simulink model "turbo_controller"  (R2025a)
settings: Solver=FixedStepAuto  StartTime=0.0  StopTime=inf  FixedStep=0.001  RelTol=1e-3
PostLoadFcn:
  | % 自动定位同目录CubeMX文件；不需要外部初始化脚本。
  | codertarget.data.setParameterValue('turbo_controller','STM32CubeMX.ProjectFile',fullfile(fileparts(get_param('turbo_controller','FileName')),'turbo_f407.ioc'));
InitFcn:
  | % 中文说明：按原控制器字段与类型创建三组接口总线；控制参数已内嵌。
  | tc_names=["EValve_Cycle" "EValve_Open" "Eblast_Cycle" "Eblast_Open" "Motor_Cycle" "Motor_Open" "EValve_Enable" "Eblast_Enable" "Motor_Enable" "SWO_Firework" "SWO_BleedAir" "EngineState" "Flag_ECUReset_Clear" "Flag_ECUReset_Save" "Flag_Reset_Enable" "Accelerator" "Nc_dem" "Nc"]; tc_types=["uint16" "uint16" "uint16" "uint16" "uint16" "uint16" "uint8" "uint8" "uint8" "uint8" "uint8" "uint8" "uint8" "uint8" "uint8" "single" "single" "single"];
  | for tc_k=1:numel(tc_names)
  |  tc_e(tc_k)=Simulink.BusElement; tc_e(tc_k).Name=char(tc_names(tc_k)); tc_e(tc_k).DataType=char(tc_types(tc_k));
  | end
  | EngineControl_Out=Simulink.Bus; EngineControl_Out.DataScope='Exported'; EngineControl_Out.Elements=tc_e;
  | clear tc_e tc_names tc_types tc_k
  | tc_names=["savedata1" "savedata2" "savedata3" "savedata4" "savedata5" "savedata6" "savedata7" "savedata8" "savedata9" "savedata10" "savedata11" "savedata12" "savedata13" "savedata14" "savedata15" "savedata16" "savedata17" "savedata18" "savedata19" "savedata20" "savedata21" "savedata22" "savedata23" "savedata24" "savedata25"]; tc_types=["single" "single" "single" "single" "single" "single" "single" "single" "single" "single" "single" "single" "single" "single" "single" "single" "single" "single" "single" "single" "single" "single" "single" "single" "single"];
  | for tc_k=1:numel(tc_names)
  |  tc_e(tc_k)=Simulink.BusElement; tc_e(tc_k).Name=char(tc_names(tc_k)); tc_e(tc_k).DataType=char(tc_types(tc_k));
  | end
  | SaveData_Out=Simulink.Bus; SaveData_Out.DataScope='Exported'; SaveData_Out.Elements=tc_e;
  | clear tc_e tc_names tc_types tc_k
  | tc_names=["senddata1" "senddata2" "senddata3" "senddata4" "senddata5" "senddata6" "senddata7" "senddata8" "senddata9" "senddata10" "senddata11" "senddata12" "senddata13" "senddata14" "senddata15" "senddata16" "senddata17" "senddata18" "senddata19" "senddata20" "senddata21" "senddata22" "senddata23" "senddata24" "senddata25" "senddata26" "senddata27" "senddata28" "senddata29"]; tc_types=["uint8" "uint8" "uint8" "uint8" "uint8" "uint8" "uint8" "uint8" "uint8" "uint8" "uint8" "uint8" "uint8" "uint8" "uint8" "uint8" "uint8" "uint8" "uint8" "uint8" "uint8" "uint8" "uint8" "uint8" "uint8" "uint8" "uint8" "uint8" "uint8"];
  | for tc_k=1:numel(tc_names)
  |  tc_e(tc_k)=Simulink.BusElement; tc_e(tc_k).Name=char(tc_names(tc_k)); tc_e(tc_k).DataType=char(tc_types(tc_k));
  | end
  | SendData_Out=Simulink.Bus; SendData_Out.DataScope='Exported'; SendData_Out.Elements=tc_e;
  | clear tc_e tc_names tc_types tc_k
  | 
  | % 以下为接口中文说明；只设置描述，不改变数值或数据类型。
  | EngineControl_Out.Description='执行控制输出（阀、电机、点火、状态及复位请求）';
  | tc_cn=["EValve_Cycle（主油阀周期计数（每计数2毫秒））" "EValve_Open（主油阀开通计数（每计数2毫秒））" "Eblast_Cycle（副油阀周期计数（每计数2毫秒））" "Eblast_Open（副油阀开通计数（每计数2毫秒））" "Motor_Cycle（起动电机周期计数）" "Motor_Open（起动电机开通计数）" "EValve_Enable（主油阀驱动使能）" "Eblast_Enable（副油阀驱动使能）" "Motor_Enable（起动电机使能）" "SWO_Firework（点火器使能（1开））" "SWO_BleedAir（引气阀使能（1开））" "EngineState（发动机状态）" "Flag_ECUReset_Clear（清除复位恢复状态请求）" "Flag_ECUReset_Save（保存复位恢复数据请求）" "Flag_Reset_Enable（处理器软件复位请求）" "Accelerator（油门／油泵给定控制量）" "Nc_dem（控制目标转速）" "Nc（发动机反馈转速（转每分））"];
  | tc_elements=EngineControl_Out.Elements;
  | for tc_k=1:numel(tc_cn)
  |  tc_elements(tc_k).Description=char(tc_cn(tc_k));
  | end
  | EngineControl_Out.Elements=tc_elements;
  | clear tc_cn tc_elements tc_k
  | SaveData_Out.Description='25项运行记录；字段含义按当前模型数据来源解释';
  | tc_cn=["savedata1（指令回显记录）" "savedata2（入口总温记录（℃））" "savedata3（电源电压记录）" "savedata4（排气温度记录（℃））" "savedata5（标定燃油压力记录）" "savedata6（副油阀占空比记录（％））" "savedata7（主油阀占空比记录（％））" "savedata8（温度修正转速记录）" "savedata9（开关输出及反馈位域）" "savedata10（物理转速记录）" "savedata11（油泵目标给定原始值）" "savedata12（起动电机占空比记录（％））" "savedata13（发动机状态码记录）" "savedata14（故障告警位域记录）" "savedata15（模型记录帧序号）" "savedata16（处理器温度记录（℃））" "savedata17（装订转速记录（沿用旧电源字段名））" "savedata18（导航高度记录）" "savedata19（飞行空速记录）" "savedata20（主阀旧记录位（恒零保留））" "savedata21（第21项保留记录（恒零））" "savedata22（保留记录项22）" "savedata23（保留记录项23）" "savedata24（保留记录项24）" "savedata25（保留记录项25）"];
  | tc_elements=SaveData_Out.Elements;
  | for tc_k=1:numel(tc_cn)
  |  tc_elements(tc_k).Description=char(tc_cn(tc_k));
  | end
  | SaveData_Out.Elements=tc_elements;
  | clear tc_cn tc_elements tc_k
  | SendData_Out.Description='29字段回传及外设命令接口；板端上位机帧只取第3至27字段';
  | tc_cn=["senddata1（回传发送允许标志（不直接上线路））" "senddata2（回传载荷长度25字节）" "senddata3（回传指令回显字节）" "senddata4（总温编码字节（℃＋80））" "senddata5（电源电压编码字节）" "senddata6（排温编码高字节）" "senddata7（排温编码低字节）" "senddata8（燃油压力编码高字节）" "senddata9（燃油压力编码低字节）" "senddata10（副油阀占空比字节（％））" "senddata11（主油阀占空比字节（％））" "senddata12（修正转速编码高字节）" "senddata13（修正转速编码低字节）" "senddata14（驱动及反馈状态位域）" "senddata15（物理转速编码高字节）" "senddata16（物理转速编码低字节）" "senddata17（油泵目标给定高字节（串口二使用））" "senddata18（油泵目标给定低字节（串口二使用））" "senddata19（起动电机占空比命令（串口一使用））" "senddata20（发动机状态码字节）" "senddata21（故障告警位域字节）" "senddata22（帧序号占位（板端另行填写））" "senddata23（处理器温度编码（℃＋50））" "senddata24（控制目标转速编码高字节）" "senddata25（控制目标转速编码低字节）" "senddata26（占位字节（板端改填实测泵速高字节））" "senddata27（占位字节（板端改填实测泵速低字节））" "senddata28（装订转速高字节（本板未发送））" "senddata29（装订转速低字节（本板未发送））"];
  | tc_elements=SendData_Out.Elements;
  | for tc_k=1:numel(tc_cn)
  |  tc_elements(tc_k).Description=char(tc_cn(tc_k));
  | end
  | SendData_Out.Elements=tc_elements;
  | clear tc_cn tc_elements tc_k
  | 
  | 
  | % FRAM模块化事务：接口类型和上电初始状态，随模型保存，无外部初始化文件。
  | clear FM_elements
  | FM_elements(1)=Simulink.BusElement;FM_elements(1).Name='phase';FM_elements(1).DataType='uint8';FM_elements(1).Dimensions=[1 1];FM_elements(1).Description='phase（当前事务阶段）';
  | FM_elements(2)=Simulink.BusElement;FM_elements(2).Name='a';FM_elements(2).DataType='uint8';FM_elements(2).Dimensions=[64 1];FM_elements(2).Description='a（启动时缓存的首区64字节）';
  | FM_elements(3)=Simulink.BusElement;FM_elements(3).Name='active';FM_elements(3).DataType='uint16';FM_elements(3).Dimensions=[1 1];FM_elements(3).Description='active（当前有效记录区地址）';
  | FM_elements(4)=Simulink.BusElement;FM_elements(4).Name='generation';FM_elements(4).DataType='uint32';FM_elements(4).Dimensions=[1 1];FM_elements(4).Description='generation（当前有效记录代号）';
  | FM_elements(5)=Simulink.BusElement;FM_elements(5).Name='record';FM_elements(5).DataType='uint8';FM_elements(5).Dimensions=[64 1];FM_elements(5).Description='record（本次冻结的待写记录）';
  | FM_elements(6)=Simulink.BusElement;FM_elements(6).Name='addr';FM_elements(6).DataType='uint16';FM_elements(6).Dimensions=[1 1];FM_elements(6).Description='addr（本次备用写入地址）';
  | FM_elements(7)=Simulink.BusElement;FM_elements(7).Name='lastSave';FM_elements(7).DataType='single';FM_elements(7).Dimensions=[1 1];FM_elements(7).Description='lastSave（上次开始保存的秒数）';
  | FM_elements(8)=Simulink.BusElement;FM_elements(8).Name='lastState';FM_elements(8).DataType='uint8';FM_elements(8).Dimensions=[1 1];FM_elements(8).Description='lastState（上次保存时的发动机状态）';
  | FM_elements(9)=Simulink.BusElement;FM_elements(9).Name='boot';FM_elements(9).DataType='boolean';FM_elements(9).Dimensions=[1 1];FM_elements(9).Description='boot（启动记录是否允许恢复）';
  | FM_elements(10)=Simulink.BusElement;FM_elements(10).Name='consumed';FM_elements(10).DataType='boolean';FM_elements(10).Dimensions=[1 1];FM_elements(10).Description='consumed（本次启动恢复通知是否已发送）';
  | FM_elements(11)=Simulink.BusElement;FM_elements(11).Name='payload';FM_elements(11).DataType='uint8';FM_elements(11).Dimensions=[20 1];FM_elements(11).Description='payload（当前20字节恢复内容）';
  | ... (+35 lines)
model workspace (MAT data in the model file):
  CRC16_Table_Reference = [0 4129 8258 12387 16516 20645 24774 28903 33032 37161 41290 45419 ... (256 elements, 256x1)]
  PE_Kaer = [0.15402 0.15402 0.12264 0.10076 0.09481 0.07601 0.07111 0.0569 0.05198 0.04926 0.05308 0.04325 ... (13 elements, 1x13)]
  PE_Nr = [21.2982 61.4260372 67.7475458 72.7394382 76.845934 80.6988798 83.8449282 86.6491912 88.9382406 89.178606 91.1938214 93.4068058 ... (13 elements, 1x13)]
  PE_Pump_Translate = 33.5999984741
  PE_RotaSpeed_Translate = 860
  PE_Taer = [0.4939154 0.4939154 0.40780982 0.34066978 0.31622756 0.30405716 0.34300244 0.26785022 0.37393554 0.23914836 0.44563948 0.31044662 ... (13 elements, 1x13)]
  PF_ACCFULLRANGE = 3360
  PF_Flag_ECUReset = 0
  PF_Flag_rx_suc = 1
  PF_Gear_Info = [40000; 45000; 50000; 55000; 57000; 59000; 60000; 61000; 61000; 61000; 61000; 61000]
  PF_K_TiaoJie = 1
  PF_Kpu = 10
  PF_MySet_Rxdata = [0 0 0 0 0 0 0 0 0 0 0 0 ... (50 elements, 50x1)]
  PF_MyUsart1_Rxdata = [0 0 0 0 0 0 0 0 0 0 0 0 ... (50 elements, 50x1)]
  PF_MyUsart2_Rxdata = [0 0 0 0 0 0 0 0 0 0 0 0 ... (50 elements, 50x1)]
  PF_Reset_Information = [0 0 0 0 0 0 0 0 0 0 0 0 ... (20 elements, 20x1)]
  PF_Sensor_X1_T4 = [0 4095]
  PF_Sensor_X2_T4 = [0 1.66666698456]
  PF_Sensor_X3_T4 = [0 504 999 1497 2010 2529 3051 3568 4076 4571 4959]
  PF_Sensor_X_P2 = [0.5 3]
  PF_Sensor_X_Poil = [0.5 3]
  PF_Sensor_X_T1t = [-50 300]
  PF_Sensor_X_Vpower = [0 3]
  PF_Sensor_X_Vpump = [0 3]
  PF_Sensor_Y1_T4 = [0 3]
  PF_Sensor_Y2_T4 = [0 5000]
  PF_Sensor_Y3_T4 = [0 100 200 300 400 500 600 700 800 900 980]
  PF_Sensor_Y_P2 = [0 1000]
  PF_Sensor_Y_Poil = [0 1000]
  PF_Sensor_Y_T1t = [-50 300]
  PF_Sensor_Y_Vpower = [0 33]
  PF_Sensor_Y_Vpump = [0 33]
  PG_CtrlMode_CloseLoop : mpt.Parameter (value not decoded)
  PG_CtrlMode_ManualAcc : mpt.Parameter (value not decoded)
  PG_CtrlMode_Origin : mpt.Parameter (value not decoded)
  PG_CtrlMode_Start : mpt.Parameter (value not decoded)
  PG_CtrlMode_Stop : mpt.Parameter (value not decoded)
  PG_ES_Clp : mpt.Parameter (value not decoded)
  PG_ES_EngStart : mpt.Parameter (value not decoded)
  PG_ES_Manual : mpt.Parameter (value not decoded)
  PG_ES_Origin : mpt.Parameter (value not decoded)
  PG_ES_Stop : mpt.Parameter (value not decoded)
  PG_Instr_BleedAirSet : mpt.Parameter (value not decoded)
  PG_Instr_CloseLoop : mpt.Parameter (value not decoded)
  PG_Instr_ECUReSet : mpt.Parameter (value not decoded)
  PG_Instr_EValveSet : mpt.Parameter (value not decoded)
  PG_Instr_EblastSet : mpt.Parameter (value not decoded)
  PG_Instr_Erase : mpt.Parameter (value not decoded)
  PG_Instr_FireWorkSet : mpt.Parameter (value not decoded)
  PG_Instr_ManualPlus : mpt.Parameter (value not decoded)
  PG_Instr_ManualrReduce : mpt.Parameter (value not decoded)
  PG_Instr_MotorSet : mpt.Parameter (value not decoded)
  PG_Instr_OilSet : mpt.Parameter (value not decoded)
  PG_Instr_SelfCheck : mpt.Parameter (value not decoded)
  PG_Instr_Start : mpt.Parameter (value not decoded)
  PG_Instr_Stop : mpt.Parameter (value not decoded)
  PG_Instr_StopZero : Simulink.Parameter (value not decoded)
  PG_Location_Air : Simulink.Parameter (value not decoded)
  PG_Location_Gnd : Simulink.Parameter (value not decoded)
  PG_ServoCtrlMode_CloseLoop : Simulink.Parameter (value not decoded)
  PG_ServoCtrlMode_CloseLoopMax : Simulink.Parameter (value not decoded)
  PG_ServoCtrlMode_CloseLoopMin : Simulink.Parameter (value not decoded)
  PG_ServoCtrlMode_ManualAcc : Simulink.Parameter (value not decoded)
  PG_ServoCtrlMode_ManualAccMax : Simulink.Parameter (value not decoded)
  PG_ServoCtrlMode_ManualAccMin : Simulink.Parameter (value not decoded)
  PG_SpeedDot_Permit : Simulink.Parameter (value not decoded)
  PL_EngineModel_Actuator = [0 10 100]
  PL_EngineModel_EngineStar_Press_P2 = [1013 1098.4 1099.144828 1099.931034 1103.613793 1162.662069 1143.793103 1131.006897 1123.186207 1117.6 1114 1111.806897 ... (127 elements, 1x127)]
  PL_EngineModel_EngineStar_RotaSpeed = [200 2000 9584 9660 10220 10240 10260 10288 10308 10368 10380 10408 ... (127 elements, 1x127)]
  PL_EngineModel_EngineStar_Temp_Exhaust = [128 129 129.1 130 131 131.1 132 133 134 134.1 135 135.1 ... (127 elements, 1x127)]
  PL_EngineModel_EngineStar_Time = [0.05 0.1 0.15 0.2 0.25 0.3 0.35 0.4 0.45 0.5 0.55 0.6 ... (127 elements, 1x127)]
  PL_EngineModel_IdleAbove_Nr = [0 21.2982 61.4260372 67.7475458 72.7394382 76.845934 80.6988798 83.8449282 86.6491912 88.9382406 89.178606 91.1938214 ... (14 elements, 1x14)]
  PL_EngineModel_IdleAbove_P2r = [0.986923266716 1.57907722675 1.81593881076 1.99358499877 2.23044658278 2.43770046879 2.65482358747 2.84233900814 3.03972366149 3.18776215149 3.25684678016 3.3950160375 ... (14 elements, 1x14)]
  PL_EngineModel_IdleAbove_Tempr = [0.0536001429337 1.07200285867 1.63301768805 1.63659103091 1.66875111667 1.72592460247 1.77595140254 1.86171163123 1.95461854565 2.03323208862 2.03323208862 2.13685903162 ... (14 elements, 1x14)]
  PL_EngineModel_IdleAbove_Ter = [0.42434128 0.42434128 0.42434128 0.30669408 0.23570008 0.22150128 0.1997974 0.23803274 0.16115638 0.24279948 0.13600422 0.31308354 ... (14 elements, 1x14)]
  PL_EngineModel_IdleAbove_Wfr = [0 10.142 23.8337 27.8905 31.9473 36.0041 40.0609 44.1177 48.1745 52.2313 52.7384 56.7952 ... (14 elements, 1x14)]
  PL_EngineModel_Press_P2 = [400 400 400 400 400 400 400 400 400 400]
  PL_EngineModel_Rotaspeed = [0 20000 96400]
  PL_EngineModel_Temp_Exhaust = [500 500 500 500 500 500 500 500 500 500]
  PL_Kaer = [0.1 0.1 0.1 0.1 0.1 0.1]
  PL_Nr = [50 60 70 80 90 100]
  PL_Taer = [0.1 0.1 0.1 0.1 0.1 0.1]
  Sig : Simulink.Signal (value not decoded)
  Ts_ms : Simulink.Parameter (value not decoded)
  false : Simulink.Parameter (value not decoded)
  true : Simulink.Parameter (value not decoded)
symbols that are objects in the model workspace (value not decoded): PG_CtrlMode_CloseLoop, PG_CtrlMode_ManualAcc, PG_CtrlMode_Origin, PG_CtrlMode_Start, PG_CtrlMode_Stop, PG_ES_Clp, PG_ES_EngStart, PG_ES_Manual, PG_ES_Origin, PG_ES_Stop, PG_Instr_BleedAirSet, PG_Instr_CloseLoop, PG_Instr_EblastSet, PG_Instr_ECUReSet, PG_Instr_Erase, PG_Instr_EValveSet, PG_Instr_FireWorkSet, PG_Instr_ManualPlus, PG_Instr_ManualrReduce, PG_Instr_MotorSet, PG_Instr_OilSet, PG_Instr_SelfCheck, PG_Instr_Start, PG_Instr_Stop, PG_Instr_StopZero, PG_ServoCtrlMode_CloseLoop, PG_ServoCtrlMode_CloseLoopMax, PG_ServoCtrlMode_CloseLoopMin, PG_ServoCtrlMode_ManualAcc, PG_ServoCtrlMode_ManualAccMax, PG_ServoCtrlMode_ManualAccMin, Ts_ms
libraries: simulink x97, stm32blockslib x10, stm32f4xxblockslib x8
(part 4 of 26)

== system turbo_controller/FRAM_复位恢复事务 ==
  note: 详细中文说明（1/1）
      | turbo_controller:536360
      | 【中文学习说明】Step01_Check（检查双区记录）
      | 一、它是做什么的？
      | 相当于检查两本备忘录有没有缺页。取67字节SPI返回帧中的第4～67字节作为64字节记
      | 录，检查记录头、提交标记和CRC32（32位校验）。输出两区是否有效、代号和恢复内
      | 容；只在相关事务阶段检查，不直接决定控制动作。
      | 二、输入和输出怎么理解？
      | 输入接口：
      | 第1路 state（上一周期事务状态）。
      | 第2路 rx（上一周期读回的67字节）。
      | 输出接口：
      | 第1路 checked（检查结果）。
      | 三、内部怎样一步步处理？
      | 01：检查读回来的记录，只判断“数据靠不靠谱”，不决定控制动作。
      | state（上一周期事务状态）：a 是启动时缓存的首区记录，phase 是当前阶段。
      | rx（上一周期读回的67字节）：前3字节是命令头，后64字节才是记录。
      | checked（检查结果）：有效标志、代号、恢复数据，以及本次原始记录。
      | 只在启动选择或写后回读阶段计算CRC，避免每毫秒重复校验。
      | 阶段17：刚完成一次写入，只校验本次回读的备用区。
      | valid（是否有效）：记录头、提交标志、CRC32三项必须同时正确。
      | [69 67 82 49] 对应记录格式标识 ECR1（复位恢复记录第1版）。
      | value（32位整数）；bytes（低字节在前的4个字节）。
      | crc（CRC32校验值）：用于检测记录内容是否损坏。
      | 四、时间、记忆与容易看错的地方
      | 学习顺序：先认本页任务与接口，再追踪条件和候选值，最后看输出来源。本文仅为说
      | 明，数值阈值、执行顺序和控制动作均由原图及参数决定。
  note: 详细中文说明（1/1）
      | turbo_controller:536361
      | 【中文学习说明】Step02_Select（选择启动恢复记录）
      | 一、它是做什么的？
      | 从上一步确认的两份记录中挑选一份。首区有效且代号不小于次区时选首区；否则若次
      | 区有效则选次区；都无效则不提供有效恢复记录。同代号优先首区。是否发出启动恢复
      | 通知还要检查记录内容的恢复资格。
      | 二、输入和输出怎么理解？
      | 输入接口：
      | 第1路 checked（检查结果）。
      | 输出接口：
      | 第1路 startup（启动选择结果）。
      | 三、内部怎样一步步处理？
      | 02：从两份已经检查过的记录中，挑出可以用于启动恢复的一份。
      | checked（双区检查结果）由01模块提供；本模块不直接访问FRAM。
      | startup（启动选择结果）：valid有效、active地址、generation代号、
      | payload恢复内容、boot是否允许发出恢复通知。
      | 首区有效且不比次区旧时，选首区；代号相同时也优先选首区。
      | 保存状态为3或4，才允许通知后面的控制逻辑进行复位恢复。
      | 四、时间、记忆与容易看错的地方
      | 学习顺序：先认本页任务与接口，再追踪条件和候选值，最后看输出来源。本文仅为说
      | 明，数值阈值、执行顺序和控制动作均由原图及参数决定。
  note: 详细中文说明（1/1）
      | turbo_controller:536362
      | 【中文学习说明】Step03_Request（判断是否开始保存）
      | 一、它是做什么的？
      | 回答“这一毫秒要不要开始保存”。必须处于空闲阶段10，并收到保存或清除请求；还
      | 要满足距离上次保存至少0.5秒，或者发动机状态已改变。只产生一个开始保存事件，
      | 不在这里写FRAM。
      | 二、输入和输出怎么理解？
      | 输入接口：
      | 第1路 state（上一周期事务状态）。
      | 第2路 control（执行控制总线）。
      | 第3路 seconds（当前秒数）。
      | 输出接口：
      | 第1路 saveEvent（本周期开始保存）。
      | 三、内部怎样一步步处理？
      | 03：只回答一个问题——“这一毫秒要不要开始保存？”
      | state（事务状态）；control（执行控制总线）；seconds（当前秒数）。
      | saveEvent（本周期开始保存）：只在空闲阶段10产生。
      | 请求来自 Flag_ECUReset_Save（保存请求）或 Flag_ECUReset_Clear（清除请求）。
      | 普通重复保存至少间隔0.5秒；发动机状态改变时允许提前保存。
      | 四、时间、记忆与容易看错的地方
      | 学习顺序：先认本页任务与接口，再追踪条件和候选值，最后看输出来源。本文仅为说
      | 明，数值阈值、执行顺序和控制动作均由原图及参数决定。
  note: 详细中文说明（1/1）
      | turbo_controller:536363
      | 【中文学习说明】Step04_Pack（打包本次运行记录）
      | 一、它是做什么的？
      | 在开始保存事件到来时，将本次运行信息冻结为20字节恢复内容，再组成带代号、头部
      | 、校验和提交信息的64字节记录。没有开始事件时不重复组包和校验。这里只整理数据
      | ，不发送SPI命令，也不推进事务阶段。
      | 二、输入和输出怎么理解？
      | 输入接口：
      | 第1路 state（上一周期事务状态）。
      | 第2路 control（执行控制总线）。
      | 第3路 send（回传协议）。
      | 第4路 data（运行记录总线）。
      | 第5路 saveEvent（本周期开始保存）。
      | 输出接口：
      | 第1路 payload（20字节恢复内容）。
      | 第2路 record（64字节完整记录）。
      | 三、内部怎样一步步处理？
      | 04：把运行状态整理成“20字节恢复内容”和“64字节完整记录”。
      | state（上一周期状态）；control（执行控制）；send（回传协议）；
      | data（运行记录总线）；saveEvent（本周期开始保存）。
      | 本模块只组装数据，不操作SPI，也不推进事务阶段。
      | 一、填写恢复内容。所有字段均明确转换成字节。
      | 第3～6、17、20字节保留为零，保持原有恢复格式。
      | 二、填写恢复内容自身的校验。
      | 三、填写完整记录头、递增代号、恢复内容及CRC32。
      | 第64字节暂时为0；必须等数据写完，再由06模块单独写165完成提交。
      | bytes（3字节数组）；value（待编码整数）；保留最低24位。
      | 四、时间、记忆与容易看错的地方
      | 学习顺序：先认本页任务与接口，再追踪条件和候选值，最后看输出来源。本文仅为说
      | 明，数值阈值、执行顺序和控制动作均由原图及参数决定。
  note: 详细中文说明（1/1）
      | turbo_controller:536364
      | 【中文学习说明】Step05_Update（推进事务并更新状态）
      | 一、它是做什么的？
      | 事务的进度管理员。启动0→读首区，1→读次区，2→选择；10等待请求。保存时按11
      | 失效标记、12写使能、13写数据、14再写使能、15提交、16回读、17核对推进。核对成
      | 功后再更新有效区信息；失败计数和一次性恢复通知也由这里管理。
      | 二、输入和输出怎么理解？
      | 输入接口：
      | 第1路 state（上一周期事务状态）。
      | 第2路 control（执行控制总线）。
      | 第3路 seconds（当前秒数）。
      | 第4路 checked（检查结果）。
      | 第5路 startup（启动选择结果）。
      | 第6路 saveEvent（本周期开始保存）。
      | 第7路 payload（20字节恢复内容）。
      | 第8路 record（64字节完整记录）。
      | 输出接口：
      | 第1路 next（下一周期状态）。
      | 第2路 restore（仅一次的恢复通知）。
      | 第3路 info（20字节恢复信息）。
      | 第4路 errors（失败计数）。
      | 三、内部怎样一步步处理？
      | 05：事务调度员。只更新状态，不组包、不计算CRC、不直接操作SPI。
      | state（上一周期状态）由00状态记忆提供；next（下一周期状态）写回00。
      | checked（01检查结果）；startup（02启动选择）；saveEvent（03保存事件）；
      | payload、record（04准备的新数据）；control（控制总线）；seconds（当前秒数）
      | 。
      | restore（仅一次的恢复通知）、info（20字节恢复信息）、errors（失败计数）。
      | 阶段表：0读首区→1读次区→2选择→10等待请求；
      | 11失效→12写使能→13写数据→14写使能→15提交→16回读→17核对。
      | 启动恢复通知只发一次，并对齐到20毫秒边界。
      | 四、时间、记忆与容易看错的地方
      | 学习顺序：先认本页任务与接口，再追踪条件和候选值，最后看输出来源。本文仅为说
      | 明，数值阈值、执行顺序和控制动作均由原图及参数决定。
  note: 详细中文说明（1/1）
      | turbo_controller:536365
      | 【中文学习说明】Step06_Command（生成分步读写命令）
      | 一、它是做什么的？
      | 将当前事务阶段翻译成SPI发送内容和发送许可。长帧67字节用于读写完整记录，4字节
      | 短帧用于标记更新，单字节0x06用于写使能。没有对应使能就不启动该路硬件传输。这
      | 里不实现SPI驱动，外层官方模块实际收发。
      | 二、输入和输出怎么理解？
      | 输入接口：
      | 第1路 state（上一周期事务状态）。
      | 第2路 saveEvent（本周期开始保存）。
      | 输出接口：
      | 第1路 tx67（本层输出接口1，具体字段见本页连线）。
      | 第2路 en67（67字节长帧/允许发送）。
      | 第3路 tx4（上位机回传帧）。
      | 第4路 en4（4字节提交帧/允许发送）。
      | 第5路 tx1（电机指令帧）。
      | 第6路 en1（单字节写使能命令/允许发送）。
      | 三、内部怎样一步步处理？
      | 06：把当前事务阶段翻译成SPI命令；外面的官方SPI模块负责真正收发。
      | state（上一周期状态）；saveEvent（本周期开始保存）。
      | tx67/en67（67字节长帧/允许发送）；tx4/en4（4字节提交帧/允许发送）；
      | tx1/en1（单字节写使能命令/允许发送）。没有使能时不会启动硬件传输。
      | frame（67字节帧）=命令1字节＋地址2字节＋数据64字节。
      | opcode（操作码）：3读、2写；address（FRAM地址）；record（待写记录）。
      | frame（4字节帧）=写命令＋地址高字节＋地址低字节＋标记值。
      | 四、时间、记忆与容易看错的地方
      | 学习顺序：先认本页任务与接口，再追踪条件和候选值，最后看输出来源。本文仅为说
      | 明，数值阈值、执行顺序和控制动作均由原图及参数决定。
  note: 用双存储区分步保存运行快照，供复位后读取
      |
      | FRAM首区地址0x0200，次区0x0300，每区一条64字节记录。启动先读两区，检查格式头、CRC32和最后
      | 的提交标记，再选择有效且代号较新的记录。没有有效记录时不发恢复通知。
      |
      | 运行中收到保存/清除请求，且空闲、间隔达到0.5 s或模式已变化时，冻结本次快照。新记录写到备用
      | 区：先把提交字节写0，再写完整记录，最后单独把提交字节写165，回读验证成功后才切换有效区。写
      | 到一半断电时，旧有效区仍可保留。
      |
      | 六个Step分别负责检查、选择、请求、打包、推进状态和生成命令。StateMemory保存上一拍事务状态
      | ；本拍发出的SPI命令，其返回帧要到后续拍再使用，不是在一段函数里同步完成全部读写。
      |
      | 恢复内容20字节包括泵给定、发动机状态、目标/实际转速等关键字段，不是保存所有ADC通道。Errors
      | 只累计写后验证失败。恢复通知对齐20 ms边界且每次启动只发一次；下游当前恢复使用使能未接通，
      | 不能把“此处有恢复通知”当成整机已恢复执行。
  note: Step01_Check（检查双区记录）
      | 检查FRAM返回记录是否完整可信
      |
      | SPI返回67字节，前3字节是命令/地址占位，后64字节才是记录。本步骤把首区缓存和本次返回的另一
      | 区分别检查，输出各区有效性、代号及20字节恢复内容。
      |
      | 一条记录必须同时满足：前4字节为ECR1（69、67、82、49）；第64字节为165；第57～60字节的小端CR
      | C32等于对第1～56字节重新计算的CRC32。只满足其中一项不算有效。
      |
      | CRC32初值FFFFFFFF，每个输入字节与低位异或，再逐位右移，最低位为1时异或EDB88320，最后逐位取
      | 反。代号按小端还原：第1字节+第2字节×256+第3字节×65536+第4字节×16777216。
      |
      | 本步骤只给检查结果，不决定哪条更新，也不修改FRAM。选择交给Step02，写后是否接受新记录交给St
      | ep05。
  note: Step02_Select（选择启动恢复记录）
      | 从双区中选出可用于启动恢复的一条
      |
      | 两区都有效时比较记录代号，优先采用代号较大的一条；代号相同优先首区。只有一条有效就选该条；
      | 两条都无效则保持valid=false，不把随机字节用于恢复。
      |
      | 输出包括所选区地址、代号和20字节内容。首区为512（0x0200），次区为768（0x0300）。代号表示保
      | 存先后，不是发动机转速或运行模式。
      |
      | boot还要求所存状态字节为3或4才成立，这是记录恢复资格规则，不等于“所有有效记录都立即恢复”
      | 。后续Step05还要等待启动读取结束、20 ms边界且尚未通知，才发一次恢复通知。代号采用普通数值
      | 比较，没有在这里额外实现代号回绕后的新旧排序。
  note: Step03_Request（判断是否开始保存）
      | 判断这一拍是否可以开始新的保存事务
      |
      | 先检查是否存在保存或清除请求：Flag_ECUReset_Save和Flag_ECUReset_Clear任一个非零都算有请求
      | 。再检查事务是否空闲，只有phase=10才允许开始，避免前一条尚未写完就覆盖快照。
      |
      | 还要满足两个条件之一：距离上次开始保存至少0.5 s，或发动机模式与上次不同。计算为“当前秒数-
      | 上次保存秒数≥0.5”，时间单位是s，不是调用次数。
      |
      | 例：刚保存0.1 s且模式未变，本拍不保存；已过0.5 s且有请求，可以保存；模式刚变且有请求，即使
      | 不足0.5 s也可以保存。输出saveEvent是一拍的开始许可，不代表FRAM已写成功。
  note: Step04_Pack（打包本次运行记录）
      | 在开始保存时冻结关键运行量，打成带校验的记录
      |
      | 只有saveEvent为真才打包；否则输出清零占位，后续由事务状态保持真正待写记录。先形成20字节恢
      | 复内容：1～2为AA55；7～8为泵给定高、低字节；9为发动机模式；10为命令回显；11～13为目标转速
      | ；14～16为实际转速；18为前17字节模256累加和，19为异或校验。其余未赋值字段保持0。
      |
      | 泵给定先限制0～65535再拆两字节。转速用三字节高位在前，例如50000保存为0、195、80。目标来自d
      | ata.savedata17，虽然记录层部分旧名称叫电源，这条线实际传的是通信目标SpeedLoad。清除请求将
      | 保存模式写0，使其失去恢复资格，并非物理擦空整片FRAM。
      |
      | 再打成64字节外层记录：1～4为ECR1，5～8为新代号（旧代号+1，小端），9～28放20字节恢复内容，5
      | 7～60为前56字节CRC32。最后提交字节先不置165，由Step06在完整写入后单独提交。
      |
      | 这里仅生成字节数组，不执行SPI；同一次事务后续始终写这份冻结快照，避免不同阶段混入不同时刻
      | 的数据。
  note: Step05_Update（推进事务并更新状态）
      | 每拍推进一个FRAM事务阶段，并保留必要记忆
      |
      | 输入state是上一拍状态，next先完整复制它，本拍只修改当前阶段需要的字段。输出next经StateMemo
      | ry延迟，下一拍才成为新的state；因此本步骤不是一次调用就完成全部SPI操作。
      |
      | 启动阶段0→1→2：发首区读取后缓存返回，再读次区，采用Step02选出的有效记录，最后进入空闲10
      | 。
      | 空闲10：saveEvent成立时，记住本次时间、模式、内容和完整记录；当前有效首区则选次区写，反之
      | 选首区，进入11。
      | 写入11～17：先使备用区失效，再发写使能、完整记录、写使能、提交165、回读，最后等待并检查返
      | 回。具体命令由Step06按旧state生成，两者要配合阅读。
      | 验证17：只有回读记录有效且代号等于原代号+1，才把新地址设为有效区并更新代号；否则失败计数加
      | 1，保留旧有效区。两种情况最终都回空闲10。
      |
      | 恢复通知另行判断：启动读取完成、boot有效、尚未通知，且四舍五入后的毫秒时间整除20时，restor
      | e置1并锁住consumed，保证一次启动只通知一次。info输出保持的20字节内容，errors输出累计验证失
      | 败次数。阶段推进本身不等于硬件回读成功。
  note: Step06_Command（生成分步读写命令）
      | 把事务阶段翻译成实际SPI字节帧
      |
      | 本步骤只看上一拍state和开始保存事件，不在内部推进阶段。三类输出分别是67字节完整帧、4字节单
      | 字节写帧、1字节写使能命令，并各带一个发送允许。长度不同对应三路执行接口，不能混用。
      |
      | 启动phase0读0x0200，phase1读0x0300；phase11向备用区地址+63写0，使它暂时无效；phase13写64字
      | 节完整记录；phase15向地址+63写165，表示提交完成；phase16回读备用区。其他阶段对应发送允许为
      | 假。
      |
      | 完整帧=[操作码,地址高字节,地址低字节,64字节]。读操作码03，后64字节发0以产生SPI时钟；写操作
      | 码02，后64字节为冻结记录。4字节帧=[02,地址高,地址低,数值]。1字节命令06用于写使能，在saveEv
      | ent、phase12、phase14发出。
      |
      | 例如备用区0x0300，提交字节地址0x033F，提交帧为02 03 3F A5。写使能必须在相应写入前发出，不
      | 能把多个阶段当成一帧连在一起。SPI实际传输由外面的带使能子系统完成。
  Control（执行控制总线） : Inport
  Send（通信回传总线） : Inport  Port=2
  Data（运行数据总线） : Inport  Port=3
  Rx67（上一周期FRAM返回帧） : Inport  Port=4
  Seconds（当前时间秒） : Inport  Port=5
  StateMemory（上一周期事务状态） : UnitDelay  Description=唯一跨周期状态记忆。阶段、地址、代号、记录和恢复标志都在FM_State中，函数模块本身无隐藏persistent变量。  InitialCondition=FM_InitialState  SampleTime=-1  HasFrameUpgradeWarning=on
  Step01_Check（检查双区记录） : MATLAB Function  Description=|  TreatAsAtomicUnit=on
      | 检查FRAM返回记录是否完整可信
      | 
      | SPI返回67字节，前3字节是命令/地址占位，后64字节才是记录。本步骤把首区缓存和本次返回的另一区分别检查，输出各区有效性、代号及20字节恢复内容。
      | 
      | 一条记录必须同时满足：前4字节为ECR1（69、67、82、49）；第64字节为165；第57～60字节的小端CRC32等于对第1～56字节重新计算的CRC32。只满足其中一项不算有效。
      | 
      | CRC32初值FFFFFFFF，每个输入字节与低位异或，再逐位右移，最低位为1时异或EDB88320，最后逐位取反。代号按小端还原：第1字节+第2字节×256+第3字节×65536+第4字节×16777216。
      | 
      | 本步骤只给检查结果，不决定哪条更新，也不修改FRAM。选择交给Step02，写后是否接受新记录交给Step05。
  Step02_Select（选择启动恢复记录） : MATLAB Function  Description=|  TreatAsAtomicUnit=on
      | 从双区中选出可用于启动恢复的一条
      | 
      | 两区都有效时比较记录代号，优先采用代号较大的一条；代号相同优先首区。只有一条有效就选该条；两条都无效则保持valid=false，不把随机字节用于恢复。
      | 
      | 输出包括所选区地址、代号和20字节内容。首区为512（0x0200），次区为768（0x0300）。代号表示保存先后，不是发动机转速或运行模式。
      | 
      | boot还要求所存状态字节为3或4才成立，这是记录恢复资格规则，不等于“所有有效记录都立即恢复”。后续Step05还要等待启动读取结束、20 ms边界且尚未通知，才发一次恢复通知。代号采用普通数值比较，没有在这里额外实现代号回绕后的新旧排序。
  Step03_Request（判断是否开始保存） : MATLAB Function  Description=|  TreatAsAtomicUnit=on
      | 判断这一拍是否可以开始新的保存事务
      | 
      | 先检查是否存在保存或清除请求：Flag_ECUReset_Save和Flag_ECUReset_Clear任一个非零都算有请求。再检查事务是否空闲，只有phase=10才允许开始，避免前一条尚未写完就覆盖快照。
      | 
      | 还要满足两个条件之一：距离上次开始保存至少0.5 s，或发动机模式与上次不同。计算为“当前秒数-上次保存秒数≥0.5”，时间单位是s，不是调用次数。
      | 
      | 例：刚保存0.1 s且模式未变，本拍不保存；已过0.5 s且有请求，可以保存；模式刚变且有请求，即使不足0.5 s也可以保存。输出saveEvent是一拍的开始许可，不代表FRAM已写成功。
  Step04_Pack（打包本次运行记录） : MATLAB Function  Description=|  TreatAsAtomicUnit=on
      | 在开始保存时冻结关键运行量，打成带校验的记录
      | 
      | 只有saveEvent为真才打包；否则输出清零占位，后续由事务状态保持真正待写记录。先形成20字节恢复内容：1～2为AA55；7～8为泵给定高、低字节；9为发动机模式；10为命令回显；11～13为目标转速；14～16为实际转速；18为前17字节模256累加和，19为异或校验。其余未赋值字段保持0。
      | 
      | 泵给定先限制0～65535再拆两字节。转速用三字节高位在前，例如50000保存为0、195、80。目标来自data.savedata17，虽然记录层部分旧名称叫电源，这条线实际传的是通信目标SpeedLoad。清除请求将保存模式写0，使其失去恢复资格，并非物理擦空整片FRAM。
      | 
      | 再打成64字节外层记录：1～4为ECR1，5～8为新代号（旧代号+1，小端），9～28放20字节恢复内容，57～60为前56字节CRC32。最后提交字节先不置165，由Step06在完整写入后单独提交。
      | 
      | 这里仅生成字节数组，不执行SPI；同一次事务后续始终写这份冻结快照，避免不同阶段混入不同时刻的数据。
  Step05_Update（推进事务并更新状态） : MATLAB Function  Description=|  TreatAsAtomicUnit=on
      | 每拍推进一个FRAM事务阶段，并保留必要记忆
      | 
      | 输入state是上一拍状态，next先完整复制它，本拍只修改当前阶段需要的字段。输出next经StateMemory延迟，下一拍才成为新的state；因此本步骤不是一次调用就完成全部SPI操作。
      | 
      | 启动阶段0→1→2：发首区读取后缓存返回，再读次区，采用Step02选出的有效记录，最后进入空闲10。
      | 空闲10：saveEvent成立时，记住本次时间、模式、内容和完整记录；当前有效首区则选次区写，反之选首区，进入11。
      | 写入11～17：先使备用区失效，再发写使能、完整记录、写使能、提交165、回读，最后等待并检查返回。具体命令由Step06按旧state生成，两者要配合阅读。
      | 验证17：只有回读记录有效且代号等于原代号+1，才把新地址设为有效区并更新代号；否则失败计数加1，保留旧有效区。两种情况最终都回空闲10。
      | 
      | 恢复通知另行判断：启动读取完成、boot有效、尚未通知，且四舍五入后的毫秒时间整除20时，restore置1并锁住consumed，保证一次启动只通知一次。info输出保持的20字节内容，errors输出累计验证失败次数。阶段推进本身不等于硬件回读成功。
  Step06_Command（生成分步读写命令） : MATLAB Function  Description=|  TreatAsAtomicUnit=on
      | 把事务阶段翻译成实际SPI字节帧
      | 
      | 本步骤只看上一拍state和开始保存事件，不在内部推进阶段。三类输出分别是67字节完整帧、4字节单字节写帧、1字节写使能命令，并各带一个发送允许。长度不同对应三路执行接口，不能混用。
      | 
      | 启动phase0读0x0200，phase1读0x0300；phase11向备用区地址+63写0，使它暂时无效；phase13写64字节完整记录；phase15向地址+63写165，表示提交完成；phase16回读备用区。其他阶段对应发送允许为假。
      | 
      | 完整帧=[操作码,地址高字节,地址低字节,64字节]。读操作码03，后64字节发0以产生SPI时钟；写操作码02，后64字节为冻结记录。4字节帧=[02,地址高,地址低,数值]。1字节命令06用于写使能，在saveEvent、phase12、phase14发出。
      | 
      | 例如备用区0x0300，提交字节地址0x033F，提交帧为02 03 3F A5。写使能必须在相应写入前发出，不能把多个阶段当成一帧连在一起。SPI实际传输由外面的带使能子系统完成。
  Tx67（完整读写帧） : Outport
  En67（完整帧发送允许） : Outport  Port=2
  Tx4（失效或提交帧） : Outport  Port=3
  En4（提交帧发送允许） : Outport  Port=4
  Tx1（写使能命令） : Outport  Port=5
  En1（写使能发送允许） : Outport  Port=6
  Restore（一次恢复通知） : Outport  Port=7
  Info20（二十字节恢复内容） : Outport  Port=8
  Errors（写后验证失败次数） : Outport  Port=9
  wires:
  Step05_Update（推进事务并更新状态）/4(errors) -> Errors（写后验证失败次数）/1  "Errors（写后验证失败次数）"
  Step05_Update（推进事务并更新状态）/3(info) -> Info20（二十字节恢复内容）/1  "Info20（二十字节恢复内容）"
  Step05_Update（推进事务并更新状态）/2(restore) -> Restore（一次恢复通知）/1  "Restore（一次恢复通知）"
  Step06_Command（生成分步读写命令）/6(en1) -> En1（写使能发送允许）/1  "En1（写使能发送允许）"
  Step06_Command（生成分步读写命令）/5(tx1) -> Tx1（写使能命令）/1  "Tx1（写使能命令）"
  Step06_Command（生成分步读写命令）/4(en4) -> En4（提交帧发送允许）/1  "En4（提交帧发送允许）"
  Step06_Command（生成分步读写命令）/3(tx4) -> Tx4（失效或提交帧）/1  "Tx4（失效或提交帧）"
  Step06_Command（生成分步读写命令）/2(en67) -> En67（完整帧发送允许）/1  "En67（完整帧发送允许）"
  Step06_Command（生成分步读写命令）/1(tx67) -> Tx67（完整读写帧）/1  "Tx67（完整读写帧）"
  Step05_Update（推进事务并更新状态）/1(next) -> StateMemory（上一周期事务状态）/1  "NextState（留给下一周期的事务状态）"
  Step04_Pack（打包本次运行记录）/2(record) -> Step05_Update（推进事务并更新状态）/8(record)  "Record64（本次完整待写记录）"
  Step04_Pack（打包本次运行记录）/1(payload) -> Step05_Update（推进事务并更新状态）/7(payload)  "Payload20（本次二十字节恢复内容）"
  Data（运行数据总线）/1 -> Step04_Pack（打包本次运行记录）/4(data)  "Data（运行数据快照）"
  Send（通信回传总线）/1 -> Step04_Pack（打包本次运行记录）/3(send)  "Send（通信回传快照）"
  Step02_Select（选择启动恢复记录）/1(startup) -> Step05_Update（推进事务并更新状态）/5(startup)  "Startup（选中的启动记录）"
  Step01_Check（检查双区记录）/1(checked) -> Step02_Select（选择启动恢复记录）/1(checked), Step05_Update（推进事务并更新状态）/4(checked)  "Checked（启动或写后校验结果）"
  Rx67（上一周期FRAM返回帧）/1 -> Step01_Check（检查双区记录）/2(rx)  "Rx67（上一周期收到的数据）"
  [FM_SaveEvent] -> Step06_Command（生成分步读写命令）/2(saveEvent)  "FM_SaveEvent（本周期开始保存）"
  [FM_SaveEvent] -> Step05_Update（推进事务并更新状态）/6(saveEvent)  "FM_SaveEvent（本周期开始保存）"
  [FM_SaveEvent] -> Step04_Pack（打包本次运行记录）/5(saveEvent)  "FM_SaveEvent（本周期开始保存）"
  Step03_Request（判断是否开始保存）/1(saveEvent) -> [FM_SaveEvent]  "FM_SaveEvent（本周期开始保存）"
  [FM_Control] -> Step05_Update（推进事务并更新状态）/2(control)  "FM_Control（执行控制快照）"
  [FM_Control] -> Step04_Pack（打包本次运行记录）/2(control)  "FM_Control（执行控制快照）"
  [FM_Control] -> Step03_Request（判断是否开始保存）/2(control)  "FM_Control（执行控制快照）"
  Control（执行控制总线）/1 -> [FM_Control]  "FM_Control（执行控制快照）"
  [FM_State] -> Step06_Command（生成分步读写命令）/1(state)  "FM_State（事务状态）"
  [FM_State] -> Step05_Update（推进事务并更新状态）/1(state)  "FM_State（事务状态）"
  [FM_State] -> Step04_Pack（打包本次运行记录）/1(state)  "FM_State（事务状态）"
  [FM_State] -> Step03_Request（判断是否开始保存）/1(state)  "FM_State（事务状态）"
  [FM_State] -> Step01_Check（检查双区记录）/1(state)  "FM_State（事务状态）"
  StateMemory（上一周期事务状态）/1 -> [FM_State]  "FM_State（事务状态）"
  [FM_Seconds] -> Step05_Update（推进事务并更新状态）/3(seconds)  "Seconds（当前时间秒）"
  [FM_Seconds] -> Step03_Request（判断是否开始保存）/3(seconds)  "Seconds（当前时间秒）"
  Seconds（当前时间秒）/1 -> [FM_Seconds]  "Seconds（当前时间秒）"

== system turbo_controller/LogPack_运行记录列定义 ==
  note: 给运行日志规定固定的27列顺序
      |
      | 把SaveData的25项数据、当前秒数及FRAM写后验证失败次数合并为27×1的single列向量。固定列序让不
      | 同采样时刻可以按同一含义解释，不应把它当作27字节通信帧。
      |
      | 这些值仍按各自记录编码保存，并非全部是国际单位制物理量。温度、压力、转速、模式和版本字段的
      | 意义不同，部分项在SaveData中已经做过比例缩放。
      |
      | 输出到SDLog的To Workspace，仿真得到engine_log。名称中的日志/SD不表示本模块已经把数据可靠落
      | 到实际SD卡；实际存储行为由外部记录接口决定。
  Savedata（运行数据总线） : Inport
  Time（时间秒） : Inport  Port=2
  Errors（恢复错误次数） : Inport  Port=3
  Column27（27行1列记录向量） : Reshape  OutputDimensionality=Column vector (2-D)
  Errors_To_Single（错误次数转单精度） : DataTypeConversion  OutDataTypeStr=single  SaturateOnIntegerOverflow=off  RndMeth=Floor
  Pack27（按记录列顺序拼接） : Mux  Inputs=27
  Select25（选择二十五项记录） : BusSelector  OutputSignals=savedata1,savedata2,savedata3,savedata4,savedata5,savedata6,savedata7,savedata8,savedata9,savedata10,savedata11,savedata12,savedata13,savedata14,savedata15,savedata16,savedata17,savedata18,savedata19,savedata20,savedata21,savedata22,savedata23,savedata24,savedata25
  Time_To_Single（时间转单精度） : DataTypeConversion  OutDataTypeStr=single  SaturateOnIntegerOverflow=off  RndMeth=Floor
  LogVector（二十七项记录） : Outport
  wires:
  Column27（27行1列记录向量）/1 -> LogVector（二十七项记录）/1  "LogVector（二十七项记录列向量）"
  Pack27（按记录列顺序拼接）/1 -> Column27（27行1列记录向量）/1  "Log27（二十七项单精度记录）"
  Errors_To_Single（错误次数转单精度）/1 -> Pack27（按记录列顺序拼接）/27  "Errors（第27项：恢复错误次数）"
  Time_To_Single（时间转单精度）/1 -> Pack27（按记录列顺序拼接）/26  "Time（第26项：时间秒）"
  Select25（选择二十五项记录）/25 -> Pack27（按记录列顺序拼接）/25  "<savedata25>"
  Select25（选择二十五项记录）/24 -> Pack27（按记录列顺序拼接）/24  "<savedata24>"
  Select25（选择二十五项记录）/23 -> Pack27（按记录列顺序拼接）/23  "<savedata23>"
  Select25（选择二十五项记录）/22 -> Pack27（按记录列顺序拼接）/22  "<savedata22>"
  Select25（选择二十五项记录）/21 -> Pack27（按记录列顺序拼接）/21  "<savedata21>"
  Select25（选择二十五项记录）/20 -> Pack27（按记录列顺序拼接）/20  "<savedata20>"
  Select25（选择二十五项记录）/19 -> Pack27（按记录列顺序拼接）/19  "<savedata19>"
  Select25（选择二十五项记录）/18 -> Pack27（按记录列顺序拼接）/18  "<savedata18>"
  Select25（选择二十五项记录）/17 -> Pack27（按记录列顺序拼接）/17  "<savedata17>"
  Select25（选择二十五项记录）/16 -> Pack27（按记录列顺序拼接）/16  "<savedata16>"
  Select25（选择二十五项记录）/15 -> Pack27（按记录列顺序拼接）/15  "<savedata15>"
  Select25（选择二十五项记录）/14 -> Pack27（按记录列顺序拼接）/14  "<savedata14>"
  Select25（选择二十五项记录）/13 -> Pack27（按记录列顺序拼接）/13  "<savedata13>"
  Select25（选择二十五项记录）/12 -> Pack27（按记录列顺序拼接）/12  "<savedata12>"
  Select25（选择二十五项记录）/11 -> Pack27（按记录列顺序拼接）/11  "<savedata11>"
  Select25（选择二十五项记录）/10 -> Pack27（按记录列顺序拼接）/10  "<savedata10>"
  Select25（选择二十五项记录）/9 -> Pack27（按记录列顺序拼接）/9  "<savedata9>"
  Select25（选择二十五项记录）/8 -> Pack27（按记录列顺序拼接）/8  "<savedata8>"
  Select25（选择二十五项记录）/7 -> Pack27（按记录列顺序拼接）/7  "<savedata7>"
  Select25（选择二十五项记录）/6 -> Pack27（按记录列顺序拼接）/6  "<savedata6>"
  Select25（选择二十五项记录）/5 -> Pack27（按记录列顺序拼接）/5  "<savedata5>"
  Select25（选择二十五项记录）/4 -> Pack27（按记录列顺序拼接）/4  "<savedata4>"
  Select25（选择二十五项记录）/3 -> Pack27（按记录列顺序拼接）/3  "<savedata3>"
  Select25（选择二十五项记录）/2 -> Pack27（按记录列顺序拼接）/2  "<savedata2>"
  Select25（选择二十五项记录）/1 -> Pack27（按记录列顺序拼接）/1  "<savedata1>"
  Errors（恢复错误次数）/1 -> Errors_To_Single（错误次数转单精度）/1  "Errors（恢复错误次数）"
  Time（时间秒）/1 -> Time_To_Single（时间转单精度）/1  "Time（时间秒）"
  Savedata（运行数据总线）/1 -> Select25（选择二十五项记录）/1  "Savedata（运行数据总线）"

== system turbo_controller/MAM ==
  note: 生成排温、转速和供电相关的监视告警
      |
      | 读取传感器总线。滤波排温T4_Filter超过850后需要定时确认；转速超过62000 rpm也需要定时确认，
      | 两条确认时间均约2 s。这样短暂一拍越限不会立即作为持续超限输出。
      |
      | ADC换算的供电电压低于22 V参与欠压判断，这条支路没有相同的2 s持续确认。告警结果打成监视总线
      | ，供状态回传等下游使用。
      |
      | 告警标志不等于本模块已经执行停车。是否切换运行模式或修改驱动，要继续查看相关标志的实际去向
      | ；本模块自身没有直接发送油泵零命令或关闭GPIO。
  S_ServoCtrlFlag : Inport
      settings: AttributesFormatString=S_ServoCtrlFlag（油泵给定选择标志）
  S_FPM : Inport  Port=2
      settings: AttributesFormatString=S_FPM（故障处理）
  S_SPM : Inport  Port=3
      settings: AttributesFormatString=S_SPM（通信及传感器信息总线）
  EngineState : Inport  Port=4
      settings: AttributesFormatString=EngineState（发动机状态）
  Bus Creator1 : BusCreator  Inputs=6
      settings: AttributesFormatString=Bus Creator1（总线创建器1）
  Bus Selector1 : BusSelector  OutputSignals=Flag_NcFailure（转速传感器故障标志）,Lock_NcFailure（转速故障锁存）
      settings: AttributesFormatString=Bus Selector1（总线选择器1）
  Bus Selector2 : BusSelector  OutputSignals=Sensor（传感器信息总线）.T4_Filter（滤波后排气温度）,Sensor（传感器信息总线）.Nc_Filter（滤波后转速）,COMM（通信信息总线）.Flag_ECUReset_Use（复位恢复数据使用标志）,Sensor（传感器信息总线）.Vpower（电源电压）
      settings: AttributesFormatString=Bus Selector2（总线选择器2）
  Constant1 : Constant  Value=62000  OutDataTypeStr=single  SampleTime=-1
      settings: AttributesFormatString=Constant1（常量1）
  Constant2 : Constant  Value=850  OutDataTypeStr=single  SampleTime=-1
      settings: AttributesFormatString=Constant2（常量2）
  Constant3 : Constant  Value=2000  OutDataTypeStr=single  SampleTime=-1
      settings: AttributesFormatString=Constant3（常量3）
  Constant4 : Constant  Value=2000  OutDataTypeStr=single  SampleTime=-1
      settings: AttributesFormatString=Constant4（常量4）
  Data Type Conversion1 : DataTypeConversion  OutDataTypeStr=uint8  SaturateOnIntegerOverflow=off  RndMeth=Floor
      settings: AttributesFormatString=Data Type Conversion1（数据类型转换1）
  Data Type Conversion3 : DataTypeConversion  OutDataTypeStr=uint8  SaturateOnIntegerOverflow=off  RndMeth=Floor
      settings: AttributesFormatString=Data Type Conversion3（数据类型转换3）
  Relational Operator : RelationalOperator  Operator=<  OutDataTypeStr=boolean  InputSameDT=off
      settings: AttributesFormatString=Relational Operator（关系比较运算）
  Relational Operator1 : RelationalOperator  Operator=>  OutDataTypeStr=boolean  InputSameDT=off
      settings: AttributesFormatString=Relational Operator1（关系比较运算1）
  Relational Operator2 : RelationalOperator  Operator=>  OutDataTypeStr=boolean  InputSameDT=off
      settings: AttributesFormatString=Relational Operator2（关系比较运算2）
  Terminator : Terminator
      settings: AttributesFormatString=Terminator（终止未使用信号）
  Terminator2 : Terminator
      settings: AttributesFormatString=Terminator2（终止未使用信号2）
  Timmer_ms : Stateflow chart  Description=|  TreatAsAtomicUnit=on  RTWFcnName=Timmer  RTWFileName=EngineControl_Timmer
      | 确认越限是否持续达到指定时间
      | 
      | 输入越限条件成立时累计次数；不成立时按图内复位分支清除本次确认。到Time_ms/Ts_ms对应的门限后，输出持续越限标志。
      | 
      | 父级给定约2000 ms，Ts_ms=20 ms，相当于约100次连续调用。温度或转速只超过一拍后恢复，不会累计成连续2 s。该定时只用于告警确认，不改变测量值，也不对排温或转速再次滤波。
      settings: AttributesFormatString=Timmer_ms（计时器毫秒）  RTWSystemCode=Reusable function  RTWFcnNameOpts=Use subsystem name  RTWFileNameOpts=User specified
  Timmer_ms1 : Stateflow chart  Description=|  TreatAsAtomicUnit=on  RTWFcnName=Timmer  RTWFileName=EngineControl_Timmer
      | 确认越限是否持续达到指定时间
      | 
      | 输入越限条件成立时累计次数；不成立时按图内复位分支清除本次确认。到Time_ms/Ts_ms对应的门限后，输出持续越限标志。
      | 
      | 父级给定约2000 ms，Ts_ms=20 ms，相当于约100次连续调用。温度或转速只超过一拍后恢复，不会累计成连续2 s。该定时只用于告警确认，不改变测量值，也不对排温或转速再次滤波。
      settings: AttributesFormatString=Timmer_ms1（计时器毫秒1）  RTWSystemCode=Reusable function  RTWFcnNameOpts=Use subsystem name  RTWFileNameOpts=User specified
  dth = T0-288.21 : Constant  Value=22  OutDataTypeStr=single  SampleTime=-1
      settings: AttributesFormatString=dth = T0-288.21（固定常量22（旧名称不参与计算））
  S_MAlarm : Outport
      settings: AttributesFormatString=S_MAlarm（报警）
  wires:
  Bus Selector2/1 -> Relational Operator2/1  "<T4_Filter（滤波后排气温度）>"
  Constant2/1 -> Relational Operator2/2
  S_SPM/1 -> Bus Selector2/1
  Relational Operator2/1 -> Timmer_ms/1(In)
  S_FPM/1 -> Bus Selector1/1
  S_ServoCtrlFlag/1 -> Terminator/1
  EngineState/1 -> Terminator2/1
  Bus Selector2/2 -> Relational Operator1/1  "<Nc_Filter（滤波后转速）>"
  Constant1/1 -> Relational Operator1/2
  Relational Operator1/1 -> Timmer_ms1/1(In)
  Timmer_ms/1(Out) -> Bus Creator1/1  "Alarm_OverTemp（超温告警）"
  Timmer_ms1/1(Out) -> Bus Creator1/2  "Alarm_OverSpeed（超转告警）"
  Bus Creator1/1 -> S_MAlarm/1
  Constant3/1 -> Timmer_ms/2(Time_ms)
  Constant4/1 -> Timmer_ms1/2(Time_ms)
  Bus Selector1/1 -> Bus Creator1/3  "<Flag_NcFailure（转速传感器故障标志）>"
  Bus Selector2/3 -> Data Type Conversion3/1  "<Flag_ECUReset_Use（复位恢复数据使用标志）>"
  Data Type Conversion3/1 -> Bus Creator1/4  "Alarm_ECUReset（控制器复位告警）"
  Bus Selector2/4 -> Relational Operator/1  "<Vpower（电源电压）>"
  Relational Operator/1 -> Data Type Conversion1/1
  dth = T0-288.21/1 -> Relational Operator/2
  Data Type Conversion1/1 -> Bus Creator1/5  "Alarm_Vpower_Low（电源欠压告警）"
  Bus Selector1/2 -> Bus Creator1/6  "<Lock_NcFailure（转速故障锁存）>"

== system turbo_controller/SDM ==
  note: 根据运行阶段组合检测标志；当前结果未参与模式控制
      |
      | 内部包含排温检查和逻辑选择，依据初始模式、起动相关条件组合出检测结果。T4_Check比较排温是否
      | 超过100，帮助区分尚冷与已经升温的状态。
      |
      | 需要注意实际去向：S_SDM送到SendData后接Unused_SDM终止端，当前没有由这条输出进一步驱动ESM起
      | 动/停车转换。这里算出了检测量，不代表它已经参与发动机状态控制。
      |
      | 实际模式转换由ESM/Flags及StateTranslation决定。阅读本模块时应将“检测算法存在”和“检测结
      | 果被控制器使用”分开。
  S_SPM : Inport
      settings: AttributesFormatString=S_SPM（通信及传感器信息总线）
  S_EngineState : Inport  Port=2
      settings: AttributesFormatString=S_EngineState（发动机状态）
  Bus Creator2 : BusCreator  Inputs=2
      settings: AttributesFormatString=Bus Creator2（总线创建器2）
  Bus Creator3 : BusCreator  Inputs=2
      settings: AttributesFormatString=Bus Creator3（总线创建器3）
  Bus Selector : BusSelector  OutputSignals=Sensor（传感器信息总线）.T4_Filter（滤波后排气温度）,Sensor（传感器信息总线）.SWI_Firework（点火器告警反馈）
      settings: AttributesFormatString=Bus Selector（总线选择器）
  Data Type Conversion1 : DataTypeConversion  OutDataTypeStr=uint8  SaturateOnIntegerOverflow=off  RndMeth=Floor
      settings: AttributesFormatString=Data Type Conversion1（数据类型转换1）
  LogicSelection3 : Subsystem  Description=|
      | 根据条件选择两种检测结果
      | 
      | C不为0时输出T，C为0时输出F。父级用它在不同运行条件下选择相应检测结果；不把两路标志相加，也不保存上次值。
      | 
      | 本处只处理选择，具体检测阈值在T4_Check及父级比较模块中。当前整个SDM结果最终接到未使用终止端，因此此选择不会单独触发实际停车或起动。
      settings: AttributesFormatString=LogicSelection3（逻辑选择3）
  N1r_idle2 : Constant  Value=0  OutDataTypeStr=uint8  SampleTime=-1
      settings: AttributesFormatString=N1r_idle2（一级转速归一化值慢车2）
  N1r_idle3 : Constant  Value=PG_ES_Origin  OutDataTypeStr=uint8  SampleTime=-1
      settings: AttributesFormatString=N1r_idle3（一级转速归一化值慢车3）
  N1r_idle8 : Constant  Value=0  OutDataTypeStr=uint8  SampleTime=-1
      settings: AttributesFormatString=N1r_idle8（一级转速归一化值慢车8）
  N1r_idle9 : Constant  Value=0  OutDataTypeStr=uint8  SampleTime=-1
      settings: AttributesFormatString=N1r_idle9（一级转速归一化值慢车9）
  Relational Operator1 : RelationalOperator  Operator===  OutDataTypeStr=boolean  InputSameDT=off
      settings: AttributesFormatString=Relational Operator1（关系比较运算1）
  Relational Operator3 : RelationalOperator  Operator===  OutDataTypeStr=boolean  InputSameDT=off
      settings: AttributesFormatString=Relational Operator3（关系比较运算3）
  T4_Check : Subsystem  Description=|
      | 用排温是否超过100判断升温条件
      | 
      | 读取排温并与100比较，输出该比较条件供SDM组合使用。这里采用已送入本模块的温度量，不直接读取ADC计数，也不重新执行传感器标定。
      | 
      | 阈值判断仅表示温度位于门限哪一侧，没有持续2 s确认，也不是完整的点火成功识别。当前SDM输出未继续参与模式控制，不能把本标志视为已经投入的起动保护。
      settings: AttributesFormatString=T4_Check（排温传感器自检）
  S_SDM : Outport
      settings: AttributesFormatString=S_SDM（传感器自检与状态数据）
  wires:
  Bus Creator3/1 -> LogicSelection3/2(F)
  N1r_idle3/1 -> Relational Operator3/2
  S_SPM/1 -> Bus Selector/1
  Bus Creator2/1 -> LogicSelection3/3(T)
  LogicSelection3/1(Out) -> S_SDM/1
  S_EngineState/1 -> Relational Operator3/1
  Relational Operator3/1 -> LogicSelection3/1(C)
  N1r_idle2/1 -> Bus Creator3/1  "Flag_T4_Check（排温检查标志）"
  N1r_idle8/1 -> Bus Creator3/2  "Flag_Vpump_Check（油泵电压检查标志）"
  Bus Selector/1 -> T4_Check/1(In1)  "<T4_Filter（滤波后排气温度）>"
  T4_Check/1(Out1) -> Bus Creator2/1  "Flag_T4_Check（排温检查标志）"
  Relational Operator1/1 -> Data Type Conversion1/1
  N1r_idle9/1 -> Relational Operator1/2
  Data Type Conversion1/1 -> Bus Creator2/2  "Flag_Vpump_Check（油泵电压检查标志）"
  Bus Selector/2 -> Relational Operator1/1  "<SWI_Firework（点火器告警反馈）>"
